simulink library "Contact_Forces_Lib"  (R2024a)
settings: Solver=ode45  StartTime=0.0  StopTime=10.0  RelTol=1e-3  EnableMultiTasking=on
undefined symbols (not defined in the file or in its folder): b_contact, custom_param_1, custom_param_2, Extr_Data_Ring, k_contact, l_cone, length_cylinder, length_tube, mu_kinetic, mu_static, pen_exponent, pen_full_damp_F, rad_s_cone, radius_cylinder, radius_tube, v_thr, X, Y, Z
libraries: nesl_utility x197, sm_lib x115, $bdroot x72, simulink x20, fl_lib x4
(part 11 of 12)

== system Contact_Forces_Lib/3D/Sphere to Cone Force/Forces/Fn/Fn in SphF ==
  R : Inport
  FxConB : Inport  Port=2
  FyConB : Inport  Port=3
  FzConB : Inport  Port=4
  Demux : Demux  Outputs=3
  Divide3 : Product  Inputs=/*  Multiplication=Matrix(*)
  Gain : Gain  Gain=-1
  Mux1 : Mux  Inputs=3
  FySphF : Outport  VectorParamsAs1DForOutWhenUnconnected=off
  FxSphF : Outport  Port=2  VectorParamsAs1DForOutWhenUnconnected=off
  FzSphF : Outport  Port=3  VectorParamsAs1DForOutWhenUnconnected=off
  wires:
  FzConB/1 -> Mux1/3
  Gain/1 -> Demux/1
  R/1 -> Divide3/1
  Demux/1 -> FxSphF/1
  Demux/2 -> FySphF/1
  Demux/3 -> FzSphF/1
  FxConB/1 -> Mux1/1
  FyConB/1 -> Mux1/2
  Mux1/1 -> Divide3/2
  Divide3/1 -> Gain/1

== system Contact_Forces_Lib/3D/Sphere to Cone Force/Forces/Fn/Fn in TubB ==
  Fn : Inport
  azm : Inport  Port=2
  Divide1 : Product  Inputs=**
  Divide2 : Product  Inputs=**
  Gain : Gain  Gain=sinConeTh
  Gain1 : Gain  Gain=sinConeTh
  cos : Trigonometry  Operator=cos
  sin : Trigonometry
  FxConB : Outport  VectorParamsAs1DForOutWhenUnconnected=off
  FyConB : Outport  Port=2  VectorParamsAs1DForOutWhenUnconnected=off
  FzConB : Outport  Port=3  VectorParamsAs1DForOutWhenUnconnected=off
  wires:
  Gain1/1 -> FzConB/1
  Gain/1 -> Divide1/1, Divide2/1
  Fn/1 -> Gain/1, Gain1/1
  azm/1 -> cos/1, sin/1
  sin/1 -> Divide2/2
  cos/1 -> Divide1/2
  Divide1/1 -> FxConB/1
  Divide2/1 -> FyConB/1

== system Contact_Forces_Lib/3D/Sphere to Cone Force/Sensing/rad_azm_cal/rad_0 ==
  Action Port : ActionPort
  Zeros : Constant  Value=[0 0 0 0]  SampleTime=0
  F : Outport  InitialOutput=[0]  VectorParamsAs1DForOutWhenUnconnected=off
  wires:
  Zeros/1 -> F/1

== system Contact_Forces_Lib/3D/Sphere to Cone Force/Sensing/rad_azm_cal/rad_azm_cal ==
  note: vazm = (x*vy - y*vx)/(x^2+y^2)
  note: vrad = (x*vx + y*vy)/z
  note: azm = atan2(y, x)
  note: rad = sqrt(x^2+y^2)
  x : Inport
  y : Inport  Port=2
  vx : Inport  Port=3
  vy : Inport  Port=4
  Action Port : ActionPort
  Add : Sum
  Add1 : Sum  Inputs=+-
  Divide : Product  Inputs=*/
  Divide1 : Product  Inputs=*/
  Math Function : Math  Operator=square  SignedPower=on
  Math Function1 : Math  Operator=square  SignedPower=on
  Mux : Mux
  Product{,1..3} (4 alike) : Product
  Sqrt : Sqrt
  Sum : Sum
  Trigonometric Function : Trigonometry  Operator=atan2
  F : Outport  VectorParamsAs1DForOutWhenUnconnected=off
  wires:
  Math Function1/1 -> Sum/2
  Math Function/1 -> Sum/1
  Sum/1 -> Divide1/2, Sqrt/1
  Trigonometric Function/1 -> Mux/2  "azm"
  x/1 -> Trigonometric Function/2, Product/1, Product2/1, Math Function/1
  y/1 -> Trigonometric Function/1, Product1/1, Product3/1, Math Function1/1
  vx/1 -> Product3/2, Product/2
  vy/1 -> Product2/2, Product1/2
  Product/1 -> Add/1
  Product1/1 -> Add/2
  Add/1 -> Divide/1
  Sqrt/1 -> Mux/1, Divide/2  "rad"
  Divide/1 -> Mux/3  "vrad"
  Product2/1 -> Add1/1
  Product3/1 -> Add1/2
  Add1/1 -> Divide1/1
  Divide1/1 -> Mux/4  "vazm"
  Mux/1 -> F/1

== system Contact_Forces_Lib/3D/Sphere to Cone Force/Sensing/rad_azm_cal/vazmx_0 ==
  Action Port : ActionPort
  Zeros : Constant  Value=0  SampleTime=0
  F : Outport  InitialOutput=[0]  VectorParamsAs1DForOutWhenUnconnected=off
  wires:
  Zeros/1 -> F/1

== system Contact_Forces_Lib/3D/Sphere to Cone Force/Sensing/rad_azm_cal/vazmx_cal ==
  note: vazmx = (y*vz - z*vy)/(y^2+z^2)
  y : Inport
  z : Inport  Port=2
  vy : Inport  Port=3
  vz : Inport  Port=4
  Action Port : ActionPort
  Add2 : Sum  Inputs=+-
  Divide2 : Product  Inputs=*/
  Math Function1 : Math  Operator=square  SignedPower=on
  Math Function2 : Math  Operator=square  SignedPower=on
  Product4 : Product
  Product5 : Product
  Sum1 : Sum
  vazmx : Outport  VectorParamsAs1DForOutWhenUnconnected=off
  wires:
  Product4/1 -> Add2/1
  Product5/1 -> Add2/2
  Add2/1 -> Divide2/1
  vy/1 -> Product5/2
  y/1 -> Math Function1/1, Product4/1
  Math Function1/1 -> Sum1/1
  z/1 -> Product5/1, Math Function2/1
  Math Function2/1 -> Sum1/2
  Sum1/1 -> Divide2/2
  vz/1 -> Product4/2
  Divide2/1 -> vazmx/1  "vazmx"

== system Contact_Forces_Lib/3D/Sphere to Cone Force/Sensing/rad_azm_cal/vazmy_0 ==
  Action Port : ActionPort
  Zeros : Constant  Value=0  SampleTime=0
  F : Outport  InitialOutput=[0]  VectorParamsAs1DForOutWhenUnconnected=off
  wires:
  Zeros/1 -> F/1

== system Contact_Forces_Lib/3D/Sphere to Cone Force/Sensing/rad_azm_cal/vazmy_cal ==
  note: vazmy = (z*vx - x*vz)/(z^2+x^2)
  x : Inport
  z : Inport  Port=2
  vx : Inport  Port=3
  vz : Inport  Port=4
  Action Port : ActionPort
  Add3 : Sum  Inputs=+-
  Divide3 : Product  Inputs=*/
  Math Function : Math  Operator=square  SignedPower=on
  Math Function2 : Math  Operator=square  SignedPower=on
  Product6 : Product
  Product7 : Product
  Sum2 : Sum
  vazmy : Outport  VectorParamsAs1DForOutWhenUnconnected=off
  wires:
  vx/1 -> Product6/2
  x/1 -> Math Function/1, Product7/1
  Math Function/1 -> Sum2/1
  Add3/1 -> Divide3/1
  Product7/1 -> Add3/2
  Product6/1 -> Add3/1
  z/1 -> Product6/1, Math Function2/1
  Math Function2/1 -> Sum2/2
  Sum2/1 -> Divide3/2
  vz/1 -> Product7/2
  Divide3/1 -> vazmy/1  "vazmy"

== system Contact_Forces_Lib/3D/Sphere to Plane Force/Forces/Ff/SlipVel ==
  wx : Inport
  wy : Inport  Port=2
  vx : Inport  Port=3
  vy : Inport  Port=4
  Fx1 : Constant  Value=sphere_rad
  Math Function : Math  Operator=square  SignedPower=on
  Math Function1 : Math  Operator=square  SignedPower=on
  Product3 : Product
  Product4 : Product
  Sqrt : Sqrt
  Sum1 : Sum  Inputs=|++
  Sum2 : Sum  Inputs=|-+
  Sum3 : Sum  Inputs=|++
  Trigonometric Function : Trigonometry  Operator=atan2
  vabs : Outport  VectorParamsAs1DForOutWhenUnconnected=off
  alpha : Outport  Port=2  VectorParamsAs1DForOutWhenUnconnected=off
  wires:
  Sum2/1 -> Math Function1/1, Trigonometric Function/2  "slipx"
  Sum1/1 -> Math Function/1, Trigonometric Function/1  "slipy"
  Math Function1/1 -> Sum3/2
  Math Function/1 -> Sum3/1
  Sum3/1 -> Sqrt/1
  Sqrt/1 -> vabs/1
  Trigonometric Function/1 -> alpha/1
  Product4/1 -> Sum2/1
  vy/1 -> Sum1/2
  Fx1/1 -> Product4/1, Product3/2
  vx/1 -> Sum2/2
  wy/1 -> Product4/2
  Product3/1 -> Sum1/1
  wx/1 -> Product3/1

== system Contact_Forces_Lib/3D/Sphere to Plane Force Enabled/Forces/Ff/SlipVel ==
  wx : Inport
  wy : Inport  Port=2
  vx : Inport  Port=3
  vy : Inport  Port=4
  Fx1 : Constant  Value=sphere_rad
  Math Function : Math  Operator=square  SignedPower=on
  Math Function1 : Math  Operator=square  SignedPower=on
  Product3 : Product
  Product4 : Product
  Sqrt : Sqrt
  Sum1 : Sum  Inputs=|++
  Sum2 : Sum  Inputs=|-+
  Sum3 : Sum  Inputs=|++
  Trigonometric Function : Trigonometry  Operator=atan2
  vabs : Outport  VectorParamsAs1DForOutWhenUnconnected=off
  alpha : Outport  Port=2  VectorParamsAs1DForOutWhenUnconnected=off
  wires:
  wx/1 -> Product3/1
  Product3/1 -> Sum1/1
  wy/1 -> Product4/2
  vx/1 -> Sum2/2
  Fx1/1 -> Product3/2, Product4/1
  vy/1 -> Sum1/2
  Product4/1 -> Sum2/1
  Trigonometric Function/1 -> alpha/1
  Sqrt/1 -> vabs/1
  Sum3/1 -> Sqrt/1
  Math Function/1 -> Sum3/1
  Math Function1/1 -> Sum3/2
  Sum1/1 -> Trigonometric Function/1, Math Function/1  "slipy"
  Sum2/1 -> Trigonometric Function/2, Math Function1/1  "slipx"

== system Contact_Forces_Lib/3D/Sphere to Sphere Force/Ff/Check w or v non zero/Else ==
  Action Port : ActionPort
  Constant : Constant  Value=0  SampleTime=0
  Constant1 : Constant  Value=[0 0 0]  SampleTime=0
  vabs : Outport  InitialOutput=0  VectorParamsAs1DForOutWhenUnconnected=off
  vuvect : Outport  Port=2  InitialOutput=0  VectorParamsAs1DForOutWhenUnconnected=off
  wires:
  Constant1/1 -> vuvect/1
  Constant/1 -> vabs/1

== system Contact_Forces_Lib/3D/Sphere to Sphere Force/Ff/Check w or v non zero/mag v ==
  vect : Inport
  Add2 : Sum  Inputs=+++
  Demux : Demux  Outputs=3
  Math Function : Math  Operator=square  SignedPower=on
  Math Function1 : Math  Operator=square  SignedPower=on
  Math Function2 : Math  Operator=square  SignedPower=on
  Sqrt : Sqrt
  mag : Outport  VectorParamsAs1DForOutWhenUnconnected=off
  wires:
  Demux/2 -> Math Function1/1
  Demux/1 -> Math Function/1
  vect/1 -> Demux/1
  Add2/1 -> Sqrt/1
  Math Function/1 -> Add2/1
  Math Function1/1 -> Add2/2
  Sqrt/1 -> mag/1
  Demux/3 -> Math Function2/1
  Math Function2/1 -> Add2/3

== system Contact_Forces_Lib/3D/Sphere to Sphere Force/Ff/Check w or v non zero/mag w ==
  vect : Inport
  Add : Sum  Inputs=+++
  Demux : Demux  Outputs=3
  Math Function : Math  Operator=square  SignedPower=on
  Math Function1 : Math  Operator=square  SignedPower=on
  Math Function2 : Math  Operator=square  SignedPower=on
  Sqrt : Sqrt
  mag : Outport  VectorParamsAs1DForOutWhenUnconnected=off
  wires:
  Math Function2/1 -> Add/3
  Demux/3 -> Math Function2/1
  Sqrt/1 -> mag/1
  Math Function1/1 -> Add/2
  Math Function/1 -> Add/1
  Add/1 -> Sqrt/1
  vect/1 -> Demux/1
  Demux/1 -> Math Function/1
  Demux/2 -> Math Function1/1

== system Contact_Forces_Lib/3D/Sphere to Sphere Force/Ff/SlipVel/If Action Subsystem ==
  In1 : Inport
  In2 : Inport  Port=2
  Action Port : ActionPort
  Divide : Product  Inputs=/*
  Out1 : Outport  VectorParamsAs1DForOutWhenUnconnected=off
  wires:
  In1/1 -> Divide/1
  In2/1 -> Divide/2
  Divide/1 -> Out1/1

== system Contact_Forces_Lib/3D/Sphere to Sphere Force/Ff/SlipVel/mag ==
  vect : Inport
  Add2 : Sum  Inputs=+++
  Demux : Demux  Outputs=3
  Math Function : Math  Operator=square  SignedPower=on
  Math Function1 : Math  Operator=square  SignedPower=on
  Math Function2 : Math  Operator=square  SignedPower=on
  Sqrt : Sqrt
  mag : Outport  VectorParamsAs1DForOutWhenUnconnected=off
  wires:
  Demux/2 -> Math Function1/1
  Demux/1 -> Math Function/1
  vect/1 -> Demux/1
  Add2/1 -> Sqrt/1
  Math Function/1 -> Add2/1
  Math Function1/1 -> Add2/2
  Sqrt/1 -> mag/1
  Demux/3 -> Math Function2/1
  Math Function2/1 -> Add2/3

== system Contact_Forces_Lib/3D/Sphere to Tube Force/Forces/Ff/Relative vel at CP ==
  note: Calculate relative velocity at contact point between sphere and tube. Two components: about ring and along tube axis. Use magnitude to calculate friction force, atan2 retains relative magnitude and direction between the components.
  Fn : Inport
  rad : Inport  Port=2
  Pen : Inport  Port=3
  vazm : Inport  Port=4
  wzf : Inport  Port=5
  vzf : Inport  Port=6
  wxf : Inport  Port=7
  wyf : Inport  Port=8
  azm : Inport  Port=9
  Calculate vRelAxis : Subsystem
  Calculate vRelRing : Subsystem
  Follower Radius : Constant  Value=radius_sphere
  Math Function : Math  Operator=square  SignedPower=on
  Math Function1 : Math  Operator=square  SignedPower=on
  Midpt Pen : Gain  Gain=0.5
  Product1 : Product
  Sign : Signum  ZeroCross=off
  Sqrt : Sqrt
  Sum1 : Sum  Inputs=+-
  Sum3 : Sum  Inputs=|++
  Trigonometric Function : Trigonometry  Operator=atan2
  vRelAbs : Outport  VectorParamsAs1DForOutWhenUnconnected=off
  rSphtoCP : Outport  Port=2  VectorParamsAs1DForOutWhenUnconnected=off
  rCyltoCP : Outport  Port=3  VectorParamsAs1DForOutWhenUnconnected=off
  alpha : Outport  Port=4  VectorParamsAs1DForOutWhenUnconnected=off
  wires:
  Calculate vRelRing/1(rCyltoCP) -> rCyltoCP/1
  wzf/1 -> Calculate vRelRing/3(wzf)
  vazm/1 -> Calculate vRelRing/2(vazm)
  rad/1 -> Calculate vRelRing/1(rad)
  Calculate vRelRing/2(vRelRing) -> Math Function/1, Trigonometric Function/2  "vRelRing"
  wyf/1 -> Calculate vRelAxis/5(wyf)
  azm/1 -> Calculate vRelAxis/4(azm)
  vzf/1 -> Calculate vRelAxis/3(vzf)
  wxf/1 -> Calculate vRelAxis/2(wxf)
  Calculate vRelAxis/1(vRelAxis) -> Trigonometric Function/1, Math Function1/1  "vRelAxis"
  Midpt Pen/1 -> Sum1/2
  Fn/1 -> Sign/1
  Pen/1 -> Midpt Pen/1
  Follower Radius/1 -> Sum1/1
  Math Function1/1 -> Sum3/2
  Math Function/1 -> Sum3/1
  Sum3/1 -> Sqrt/1
  Sqrt/1 -> vRelAbs/1
  Trigonometric Function/1 -> alpha/1  "alpha"
  Sign/1 -> Product1/2  "InOut"
  Sum1/1 -> Product1/1, rSphtoCP/1  "rSphtoCP"
  Product1/1 -> Calculate vRelAxis/1(rSphtoCP sign), Calculate vRelRing/4(rSphtoCP sign)

== system Contact_Forces_Lib/3D/Sphere to Tube Force/Forces/Ff/Resolve Ff ==
  note: Resolve Friction Force in
      | Tube B reference frame
  note: Resolve Friction Force in
      | Sphere F reference frame
  InOut : Inport
  Ff : Inport  Port=2
  rSphtoCP : Inport  Port=3
  rCyltoCP : Inport  Port=4
  alpha : Inport  Port=5
  z : Inport  Port=6
  R : Inport  Port=7
  azm : Inport  Port=8
  Ff in SphF : Subsystem
  Ff in TubB : Subsystem
  FxSphF : Outport  VectorParamsAs1DForOutWhenUnconnected=off
  FySphF : Outport  Port=2  VectorParamsAs1DForOutWhenUnconnected=off
  FzSphF : Outport  Port=3  VectorParamsAs1DForOutWhenUnconnected=off
  TSphF : Outport  Port=4  VectorParamsAs1DForOutWhenUnconnected=off
  FxSphB : Outport  Port=5  VectorParamsAs1DForOutWhenUnconnected=off
  FyTubB : Outport  Port=6  VectorParamsAs1DForOutWhenUnconnected=off
  FzTubB : Outport  Port=7  VectorParamsAs1DForOutWhenUnconnected=off
  TTubB : Outport  Port=8  VectorParamsAs1DForOutWhenUnconnected=off
  wires:
  InOut/1 -> Ff in TubB/1(InOut)
  z/1 -> Ff in TubB/7(z)
  rSphtoCP/1 -> Ff in TubB/5(rSphtoCP)
  rCyltoCP/1 -> Ff in TubB/6(rCyltoCP)
  Ff/1 -> Ff in TubB/2(Ff)
  Ff in SphF/1(FySphF) -> FySphF/1
  Ff in TubB/1(FxTubB) -> Ff in SphF/1(FxTubB), FxSphB/1
  Ff in TubB/2(FyTubB) -> FyTubB/1, Ff in SphF/2(FyTubB)
  Ff in SphF/2(FxSphF) -> FxSphF/1
  azm/1 -> Ff in TubB/3(azm)
  R/1 -> Ff in SphF/5(R)
  Ff in SphF/3(FzSphF) -> FzSphF/1
  Ff in TubB/3(FzTubB) -> Ff in SphF/3(FzTubB), FzTubB/1
  alpha/1 -> Ff in TubB/4(alpha)
  Ff in TubB/5(TTubB) -> TTubB/1
  Ff in TubB/4(TSphF_B) -> Ff in SphF/4(TSphF_B)
  Ff in SphF/4(TSphF) -> TSphF/1

== system Contact_Forces_Lib/3D/Sphere to Tube Force/Forces/Fn/Fn in SphF ==
  R : Inport
  FxTubB : Inport  Port=2
  FyTubB : Inport  Port=3
  Constant : Constant  Value=0
  Demux : Demux  Outputs=3
  Divide3 : Product  Inputs=/*  Multiplication=Matrix(*)
  Gain : Gain  Gain=-1
  Mux1 : Mux  Inputs=3
  FySphF : Outport  VectorParamsAs1DForOutWhenUnconnected=off
  FxSphF : Outport  Port=2  VectorParamsAs1DForOutWhenUnconnected=off
  FzSphF : Outport  Port=3  VectorParamsAs1DForOutWhenUnconnected=off
  wires:
  Divide3/1 -> Gain/1
  Mux1/1 -> Divide3/2
  FyTubB/1 -> Mux1/2
  FxTubB/1 -> Mux1/1
  Demux/3 -> FzSphF/1
  Demux/2 -> FySphF/1
  Demux/1 -> FxSphF/1
  Constant/1 -> Mux1/3
  R/1 -> Divide3/1
  Gain/1 -> Demux/1

== system Contact_Forces_Lib/3D/Sphere to Tube Force/Forces/Fn/Fn in TubB ==
  Fn : Inport
  azm : Inport  Port=2
  Divide1 : Product  Inputs=**
  Divide2 : Product  Inputs=**
  cos : Trigonometry  Operator=cos
  sin : Trigonometry
  FxTubB : Outport  VectorParamsAs1DForOutWhenUnconnected=off
  FyTubB : Outport  Port=2  VectorParamsAs1DForOutWhenUnconnected=off
  wires:
  Divide2/1 -> FyTubB/1
  Divide1/1 -> FxTubB/1
  cos/1 -> Divide1/2
  sin/1 -> Divide2/2
  azm/1 -> sin/1, cos/1
  Fn/1 -> Divide2/1, Divide1/1

== system Contact_Forces_Lib/3D/Sphere to Tube Force/Sensing/rad_azm_cal/rad_0 ==
  Action Port : ActionPort
  Zeros : Constant  Value=[0 0 0 0]  SampleTime=0
  F : Outport  InitialOutput=[0]  VectorParamsAs1DForOutWhenUnconnected=off
  wires:
  Zeros/1 -> F/1

== system Contact_Forces_Lib/3D/Sphere to Tube Force/Sensing/rad_azm_cal/rad_azm_cal ==
  note: z = sqrt(x2+y2)
      | zdot = 1/z(x*xdot+y*ydot)
      | azm = atan(y/x)
      | azmdot = 1/z2(x*ydot-xdot*y)
  X : Inport
  Y : Inport  Port=2
  Xdot : Inport  Port=3
  Ydot : Inport  Port=4
  Action Port : ActionPort
  Add : Sum
  Add1 : Sum  Inputs=+-
  Divide : Product  Inputs=*/
  Divide1 : Product  Inputs=*/
  Math Function : Math  Operator=square  SignedPower=on
  Math Function1 : Math  Operator=square  SignedPower=on
  Mux : Mux
  Product{,1..3} (4 alike) : Product
  Sqrt : Sqrt
  Sum : Sum  Inputs=|++
  Trigonometric Function : Trigonometry  Operator=atan2
  F : Outport  VectorParamsAs1DForOutWhenUnconnected=off
  wires:
  Mux/1 -> F/1
  Divide1/1 -> Mux/4
  Add1/1 -> Divide1/1
  Product3/1 -> Add1/2
  Product2/1 -> Add1/1
  Divide/1 -> Mux/3
  Sqrt/1 -> Divide/2, Mux/1
  Add/1 -> Divide/1
  Product1/1 -> Add/2
  Product/1 -> Add/1
  Ydot/1 -> Product1/2, Product2/2
  Xdot/1 -> Product/2, Product3/2
  Y/1 -> Math Function1/1, Product1/1, Product3/1, Trigonometric Function/1
  X/1 -> Math Function/1, Product/1, Product2/1, Trigonometric Function/2
  Trigonometric Function/1 -> Mux/2
  Sum/1 -> Sqrt/1, Divide1/2
  Math Function/1 -> Sum/1
  Math Function1/1 -> Sum/2

== system Contact_Forces_Lib/3D/Sphere to Tube Force Enabled/Forces/Ff/Relative vel at CP ==
  note: Calculate relative velocity at contact point between sphere and tube. Two components: about ring and along tube axis. Use magnitude to calculate friction force, atan2 retains relative magnitude and direction between the components.
  Fn : Inport
  rad : Inport  Port=2
  Pen : Inport  Port=3
  vazm : Inport  Port=4
  wzf : Inport  Port=5
  vzf : Inport  Port=6
  wxf : Inport  Port=7
  wyf : Inport  Port=8
  azm : Inport  Port=9
  Calculate vRelAxis : Subsystem
  Calculate vRelRing : Subsystem
  Follower Radius : Constant  Value=radius_sphere
  Math Function : Math  Operator=square  SignedPower=on
  Math Function1 : Math  Operator=square  SignedPower=on
  Midpt Pen : Gain  Gain=0.5
  Product1 : Product
  Sign : Signum  ZeroCross=off
  Sqrt : Sqrt
  Sum1 : Sum  Inputs=+-
  Sum3 : Sum  Inputs=|++
  Trigonometric Function : Trigonometry  Operator=atan2
  vRelAbs : Outport  VectorParamsAs1DForOutWhenUnconnected=off
  rSphtoCP : Outport  Port=2  VectorParamsAs1DForOutWhenUnconnected=off
  rCyltoCP : Outport  Port=3  VectorParamsAs1DForOutWhenUnconnected=off
  alpha : Outport  Port=4  VectorParamsAs1DForOutWhenUnconnected=off
  wires:
  Calculate vRelRing/1(rCyltoCP) -> rCyltoCP/1
  wzf/1 -> Calculate vRelRing/3(wzf)
  vazm/1 -> Calculate vRelRing/2(vazm)
  rad/1 -> Calculate vRelRing/1(rad)
  Calculate vRelRing/2(vRelRing) -> Math Function/1, Trigonometric Function/2  "vRelRing"
  wyf/1 -> Calculate vRelAxis/5(wyf)
  azm/1 -> Calculate vRelAxis/4(azm)
  vzf/1 -> Calculate vRelAxis/3(vzf)
  wxf/1 -> Calculate vRelAxis/2(wxf)
  Calculate vRelAxis/1(vRelAxis) -> Trigonometric Function/1, Math Function1/1  "vRelAxis"
  Midpt Pen/1 -> Sum1/2
  Fn/1 -> Sign/1
  Pen/1 -> Midpt Pen/1
  Follower Radius/1 -> Sum1/1
  Math Function1/1 -> Sum3/2
  Math Function/1 -> Sum3/1
  Sum3/1 -> Sqrt/1
  Sqrt/1 -> vRelAbs/1
  Trigonometric Function/1 -> alpha/1  "alpha"
  Sign/1 -> Product1/2  "InOut"
  Sum1/1 -> Product1/1, rSphtoCP/1  "rSphtoCP"
  Product1/1 -> Calculate vRelAxis/1(rSphtoCP sign), Calculate vRelRing/4(rSphtoCP sign)

== system Contact_Forces_Lib/3D/Sphere to Tube Force Enabled/Forces/Ff/Resolve Ff ==
  note: Resolve Friction Force in
      | Tube B reference frame
  note: Resolve Friction Force in
      | Sphere F reference frame
  InOut : Inport
  Ff : Inport  Port=2
  rSphtoCP : Inport  Port=3
  rCyltoCP : Inport  Port=4
  alpha : Inport  Port=5
  z : Inport  Port=6
  R : Inport  Port=7
  azm : Inport  Port=8
  Ff in SphF : Subsystem
  Ff in TubB : Subsystem
  FxSphF : Outport  VectorParamsAs1DForOutWhenUnconnected=off
  FySphF : Outport  Port=2  VectorParamsAs1DForOutWhenUnconnected=off
  FzSphF : Outport  Port=3  VectorParamsAs1DForOutWhenUnconnected=off
  TSphF : Outport  Port=4  VectorParamsAs1DForOutWhenUnconnected=off
  FxSphB : Outport  Port=5  VectorParamsAs1DForOutWhenUnconnected=off
  FyTubB : Outport  Port=6  VectorParamsAs1DForOutWhenUnconnected=off
  FzTubB : Outport  Port=7  VectorParamsAs1DForOutWhenUnconnected=off
  TTubB : Outport  Port=8  VectorParamsAs1DForOutWhenUnconnected=off
  wires:
  InOut/1 -> Ff in TubB/1(InOut)
  z/1 -> Ff in TubB/7(z)
  rSphtoCP/1 -> Ff in TubB/5(rSphtoCP)
  rCyltoCP/1 -> Ff in TubB/6(rCyltoCP)
  Ff/1 -> Ff in TubB/2(Ff)
  Ff in SphF/1(FySphF) -> FySphF/1
  Ff in TubB/1(FxTubB) -> Ff in SphF/1(FxTubB), FxSphB/1
  Ff in TubB/2(FyTubB) -> FyTubB/1, Ff in SphF/2(FyTubB)
  Ff in SphF/2(FxSphF) -> FxSphF/1
  azm/1 -> Ff in TubB/3(azm)
  R/1 -> Ff in SphF/5(R)
  Ff in SphF/3(FzSphF) -> FzSphF/1
  Ff in TubB/3(FzTubB) -> Ff in SphF/3(FzTubB), FzTubB/1
  alpha/1 -> Ff in TubB/4(alpha)
  Ff in TubB/5(TTubB) -> TTubB/1
  Ff in TubB/4(TSphF_B) -> Ff in SphF/4(TSphF_B)
  Ff in SphF/4(TSphF) -> TSphF/1

== system Contact_Forces_Lib/3D/Sphere to Tube Force Enabled/Forces/Fn/Fn in SphF ==
  R : Inport
  FxTubB : Inport  Port=2
  FyTubB : Inport  Port=3
  Constant : Constant  Value=0
  Demux : Demux  Outputs=3
  Divide3 : Product  Inputs=/*  Multiplication=Matrix(*)
  Gain : Gain  Gain=-1
  Mux1 : Mux  Inputs=3
  FySphF : Outport  VectorParamsAs1DForOutWhenUnconnected=off
  FxSphF : Outport  Port=2  VectorParamsAs1DForOutWhenUnconnected=off
  FzSphF : Outport  Port=3  VectorParamsAs1DForOutWhenUnconnected=off
  wires:
  Divide3/1 -> Gain/1
  Mux1/1 -> Divide3/2
  FyTubB/1 -> Mux1/2
  FxTubB/1 -> Mux1/1
  Demux/3 -> FzSphF/1
  Demux/2 -> FySphF/1
  Demux/1 -> FxSphF/1
  Constant/1 -> Mux1/3
  R/1 -> Divide3/1
  Gain/1 -> Demux/1

== system Contact_Forces_Lib/3D/Sphere to Tube Force Enabled/Forces/Fn/Fn in TubB ==
  Fn : Inport
  azm : Inport  Port=2
  Divide1 : Product  Inputs=**
  Divide2 : Product  Inputs=**
  cos : Trigonometry  Operator=cos
  sin : Trigonometry
  FxTubB : Outport  VectorParamsAs1DForOutWhenUnconnected=off
  FyTubB : Outport  Port=2  VectorParamsAs1DForOutWhenUnconnected=off
  wires:
  Divide2/1 -> FyTubB/1
  Divide1/1 -> FxTubB/1
  cos/1 -> Divide1/2
  sin/1 -> Divide2/2
  azm/1 -> sin/1, cos/1
  Fn/1 -> Divide2/1, Divide1/1

== system Contact_Forces_Lib/3D/Sphere to Tube Force Enabled/Sensing/rad_azm_cal/rad_0 ==
  Action Port : ActionPort
  Zeros : Constant  Value=[0 0 0 0]  SampleTime=0
  F : Outport  InitialOutput=[0]  VectorParamsAs1DForOutWhenUnconnected=off
  wires:
  Zeros/1 -> F/1

== system Contact_Forces_Lib/3D/Sphere to Tube Force Enabled/Sensing/rad_azm_cal/rad_azm_cal ==
  note: z = sqrt(x2+y2)
      | zdot = 1/z(x*xdot+y*ydot)
      | azm = atan(y/x)
      | azmdot = 1/z2(x*ydot-xdot*y)
  X : Inport
  Y : Inport  Port=2
  Xdot : Inport  Port=3
  Ydot : Inport  Port=4
  Action Port : ActionPort
  Add : Sum
  Add1 : Sum  Inputs=+-
  Divide : Product  Inputs=*/
  Divide1 : Product  Inputs=*/
  Math Function : Math  Operator=square  SignedPower=on
  Math Function1 : Math  Operator=square  SignedPower=on
  Mux : Mux
  Product{,1..3} (4 alike) : Product
  Sqrt : Sqrt
  Sum : Sum  Inputs=|++
  Trigonometric Function : Trigonometry  Operator=atan2
  F : Outport  VectorParamsAs1DForOutWhenUnconnected=off
  wires:
  Mux/1 -> F/1
  Divide1/1 -> Mux/4
  Add1/1 -> Divide1/1
  Product3/1 -> Add1/2
  Product2/1 -> Add1/1
  Divide/1 -> Mux/3
  Sqrt/1 -> Divide/2, Mux/1
  Add/1 -> Divide/1
  Product1/1 -> Add/2
  Product/1 -> Add/1
  Ydot/1 -> Product1/2, Product2/2
  Xdot/1 -> Product/2, Product3/2
  Y/1 -> Math Function1/1, Product1/1, Product3/1, Trigonometric Function/1
  X/1 -> Math Function/1, Product/1, Product2/1, Trigonometric Function/2
  Trigonometric Function/1 -> Mux/2
  Sum/1 -> Sqrt/1, Divide1/2
  Math Function/1 -> Sum/1
  Math Function1/1 -> Sum/2

== system Contact_Forces_Lib/2D/Circle to Finite Line Force/Forces/Resolve Forces/Friction/VCirPt ==
  wz : Inport
  X sep : Inport  Port=2
  Constant : Constant  Value=line_depth
  Product : Product
  Product1 : Product
  Sign1 : Signum
  Subtract : Sum  Inputs=+-
  vCir : Outport  VectorParamsAs1DForOutWhenUnconnected=off
  wires:
  wz/1 -> Product1/1
  Product1/1 -> vCir/1
  Product/1 -> Subtract/2
  Sign1/1 -> Product/1
  X sep/1 -> Subtract/1, Sign1/1
  Constant/1 -> Product/2
  Subtract/1 -> Product1/2

== system Contact_Forces_Lib/2D/Circle to Finite Line Force Enabled/Forces/Resolve Forces/Friction/VCirPt ==
  wz : Inport
  X sep : Inport  Port=2
  Constant : Constant  Value=line_depth
  Product : Product
  Product1 : Product
  Sign1 : Signum
  Subtract : Sum  Inputs=+-
  vCir : Outport  VectorParamsAs1DForOutWhenUnconnected=off
  wires:
  Subtract/1 -> Product1/2
  Constant/1 -> Product/2
  X sep/1 -> Sign1/1, Subtract/1
  Sign1/1 -> Product/1
  Product/1 -> Subtract/2
  Product1/1 -> vCir/1
  wz/1 -> Product1/1

== system Contact_Forces_Lib/2D/Circle to Ring Force/Forces/Ff/Resolve Ff/Ff in CirB ==
  Ff : Inport
  azm : Inport  Port=2
  Divide1 : Product  Inputs=**
  Divide2 : Product  Inputs=**
  Gain1 : Gain
  Gain3 : Gain  Gain=-1
  cos : Trigonometry
  deg2rad : Gain  Gain=pi/180
  sin : Trigonometry  Operator=cos
  FxRinB : Outport  VectorParamsAs1DForOutWhenUnconnected=off
  FyRinB : Outport  Port=2  VectorParamsAs1DForOutWhenUnconnected=off
  wires:
  Gain1/1 -> Divide2/1, Divide1/1
  azm/1 -> deg2rad/1
  Divide2/1 -> FyRinB/1
  cos/1 -> Gain3/1
  sin/1 -> Divide2/2
  deg2rad/1 -> sin/1, cos/1
  Divide1/1 -> FxRinB/1
  Ff/1 -> Gain1/1
  Gain3/1 -> Divide1/2

== system Contact_Forces_Lib/2D/Circle to Ring Force/Forces/Ff/Resolve Ff/Ff in CirF ==
  R : Inport
  FxRinB : Inport  Port=2
  FyRinB : Inport  Port=3
  Demux : Demux  Outputs=2
  Divide3 : Product  Inputs=**  Multiplication=Matrix(*)
  Gain1 : Gain  Gain=-1
  Mux1 : Mux  Inputs=2
  FyCirF : Outport  VectorParamsAs1DForOutWhenUnconnected=off
  FxCirF : Outport  Port=2  VectorParamsAs1DForOutWhenUnconnected=off
  wires:
  R/1 -> Divide3/1
  Divide3/1 -> Gain1/1
  Mux1/1 -> Divide3/2
  Gain1/1 -> Demux/1
  Demux/1 -> FyCirF/1
  Demux/2 -> FxCirF/1
  FyRinB/1 -> Mux1/1
  FxRinB/1 -> Mux1/2

== system Contact_Forces_Lib/2D/Circle to Ring Force/Forces/Ff/Resolve Ff/Tz ==
  rCirFtoCP : Inport
  rRinBtoCP : Inport  Port=2
  Ff : Inport  Port=3
  Divide4 : Product  Inputs=**
  Divide5 : Product  Inputs=**
  Gain2 : Gain  Gain=-1
  TzRinB : Outport  VectorParamsAs1DForOutWhenUnconnected=off
  TzCirF : Outport  Port=2  VectorParamsAs1DForOutWhenUnconnected=off
  wires:
  rRinBtoCP/1 -> Divide5/2
  Divide5/1 -> TzRinB/1
  rCirFtoCP/1 -> Divide4/2
  Divide4/1 -> TzCirF/1
  Gain2/1 -> Divide5/1
  Ff/1 -> Divide4/1, Gain2/1

== system Contact_Forces_Lib/3D/Prototype/Cone in Ring Force/Point of Contact calc/Force Calc/Computing Force from nonzero penetration points ==
  Y : Inport
  X : Inport  Port=2
  Pen : Inport  Port=3
  Derivative : Derivative  Commented=on  CoefficientInTFapproximation=1e-4
  For Each Subsystem1 : Subsystem  Commented=on  TreatAsAtomicUnit=on
  For Iterator Subsystem : Subsystem  Commented=on  TreatAsAtomicUnit=on
  Gain1 : Gain  Commented=on  Gain=-1
  Linear1 : Subsystem  Commented=on  VariantControl=Linear  mask(Linear Force Law){k_pen=1e4, b_penvel=1e3}
      mask prompts: k_pen "Contact Stiffness"; b_penvel "Contact Damping"
      mask help: Implements a contact force law as a linear spring damper. The damping force is applied only as the penetration depth increases.
      mask Help: web(which('Force_Laws.html'));
  Product2 : Product  Commented=on
  Product3 : Product  Commented=on
  Sum of Elements : Sum  Commented=on  Inputs=+
  Sum of Elements1 : Sum  Commented=on  Inputs=+
  Sum3 : Sum  Commented=on  Inputs=|+-
  Trigonometric Function3 : Trigonometry  Commented=on  Operator=atan2
  Trigonometric Function4 : Trigonometry  Commented=on  Operator=cos
  Trigonometric Function5 : Trigonometry  Commented=on
  Fx : Outport  VectorParamsAs1DForOutWhenUnconnected=off
  Fy : Outport  Port=2  VectorParamsAs1DForOutWhenUnconnected=off
  wires:
  Trigonometric Function3/1 -> Trigonometric Function5/1, Trigonometric Function4/1
  Linear1/2(Damp F) -> Sum3/2
  Trigonometric Function5/1 -> Product3/1
  Trigonometric Function4/1 -> Product2/1
  Gain1/1 -> Product2/2, Product3/2
  Sum3/1 -> Gain1/1
  Linear1/1(Spr F) -> Sum3/1
  Sum of Elements1/1 -> Fy/1
  Pen/1 -> Derivative/1, For Each Subsystem1/1(In1), Linear1/1(Pen)
  X/1 -> Trigonometric Function3/2
  Y/1 -> Trigonometric Function3/1
  Sum of Elements/1 -> Fx/1
  Derivative/1 -> Linear1/2(Pen Vel)
  Product2/1 -> Sum of Elements/1
  Product3/1 -> Sum of Elements1/1

== system Contact_Forces_Lib/3D/Prototype/Cone in Ring Force/Point of Contact calc/Force Calc/MAX_ML ==
  Y : Inport
  X : Inport  Port=2
  pen : Inport  Port=3
  Gain : Gain  Gain=-1
  Linear : Subsystem  VariantControl=Linear  mask(Linear Force Law){k_pen=k_stiff, b_penvel=b_damp}
      mask prompts: k_pen "Contact Stiffness"; b_penvel "Contact Damping"
      mask help: Implements a contact force law as a linear spring damper. The damping force is applied only as the penetration depth increases.
      mask Help: web(which('Force_Laws.html'));
  MATLAB Function : MATLAB Function  TreatAsAtomicUnit=on
  Product : Product
  Product1 : Product
  Sum2 : Sum  Inputs=|+-
  Transfer Fcn : TransferFcn  Numerator=[1 0]  Denominator=[1e-4 1]
  Trigonometric Function : Trigonometry  Operator=atan2
  Trigonometric Function1 : Trigonometry  Operator=cos
  Trigonometric Function2 : Trigonometry
  Fx : Outport  VectorParamsAs1DForOutWhenUnconnected=off
  Fy : Outport  Port=2  VectorParamsAs1DForOutWhenUnconnected=off
  wires:
  Product1/1 -> Fy/1
  MATLAB Function/4(ind) -> ?
  X/1 -> MATLAB Function/2(x)
  Product/1 -> Fx/1
  pen/1 -> MATLAB Function/1(pen)
  Transfer Fcn/1 -> Linear/2(Pen Vel)
  Gain/1 -> Product1/2, Product/2
  Trigonometric Function1/1 -> Product/1
  Linear/1(Spr F) -> Sum2/1
  Trigonometric Function2/1 -> Product1/1
  Sum2/1 -> Gain/1
  Linear/2(Damp F) -> Sum2/2
  Trigonometric Function/1 -> Trigonometric Function1/1, Trigonometric Function2/1
  Y/1 -> MATLAB Function/3(y)
  MATLAB Function/2(yc) -> Trigonometric Function/1
  MATLAB Function/1(xc) -> Trigonometric Function/2
  MATLAB Function/3(penc) -> Transfer Fcn/1, Linear/1(Pen)

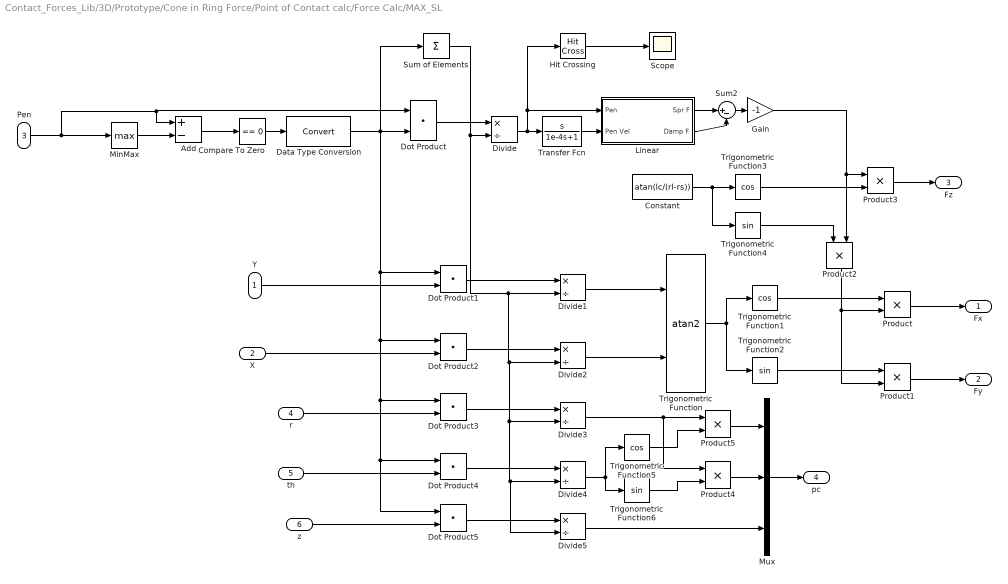
== system Contact_Forces_Lib/3D/Prototype/Cone in Ring Force/Point of Contact calc/Force Calc/MAX_SL ==
  Y : Inport
  X : Inport  Port=2
  Pen : Inport  Port=3
  r : Inport  Port=4
  th : Inport  Port=5
  z : Inport  Port=6
  Add : Sum  Inputs=+-
  Compare To Zero : simulink/Logic and Bit Operations/Compare To Zero  relop===  OutDataTypeStr=boolean  ZeroCross=off
  Constant : Constant  Value=atan(lc/(rl-rs))
  Data Type Conversion : DataTypeConversion  SaturateOnIntegerOverflow=off  RndMeth=Floor
  Divide{,1..5} (6 alike) : Product  Inputs=*/
  Dot Product{,1..5} (6 alike) : DotProduct  OutDataTypeStr=Inherit: Inherit via internal rule
  Gain : Gain  Gain=-1
  Hit Crossing : HitCross
  Linear : Subsystem  VariantControl=Linear  mask(Linear Force Law){k_pen=k_stiff, b_penvel=b_damp}
      mask prompts: k_pen "Contact Stiffness"; b_penvel "Contact Damping"
      mask help: Implements a contact force law as a linear spring damper. The damping force is applied only as the penetration depth increases.
      mask Help: web(which('Force_Laws.html'));
  MinMax : MinMax  Function=max  ZeroCross=off
  Mux : Mux  Inputs=3
  Product{,1..5} (6 alike) : Product
  Scope : Scope
  Sum of Elements : Sum  Inputs=+
  Sum2 : Sum  Inputs=|+-
  Transfer Fcn : TransferFcn  Numerator=[1 0]  Denominator=[1e-4 1]
  Trigonometric Function : Trigonometry  Operator=atan2
  Trigonometric Function1 : Trigonometry  Operator=cos
  Trigonometric Function2 : Trigonometry
  Trigonometric Function3 : Trigonometry  Operator=cos
  Trigonometric Function4 : Trigonometry
  Trigonometric Function5 : Trigonometry  Operator=cos
  Trigonometric Function6 : Trigonometry
  Fx : Outport  VectorParamsAs1DForOutWhenUnconnected=off
  Fy : Outport  Port=2  VectorParamsAs1DForOutWhenUnconnected=off
  Fz : Outport  Port=3  VectorParamsAs1DForOutWhenUnconnected=off
  pc : Outport  Port=4  VectorParamsAs1DForOutWhenUnconnected=off
  wires:
  Trigonometric Function/1 -> Trigonometric Function2/1, Trigonometric Function1/1
  Linear/2(Damp F) -> Sum2/2
  Sum2/1 -> Gain/1
  Trigonometric Function2/1 -> Product1/1
  Linear/1(Spr F) -> Sum2/1
  Trigonometric Function1/1 -> Product/1
  Transfer Fcn/1 -> Linear/2(Pen Vel)
  MinMax/1 -> Add/2
  Add/1 -> Compare To Zero/1
  Compare To Zero/1 -> Data Type Conversion/1
  Product/1 -> Fx/1
  Pen/1 -> Dot Product/1, Add/1, MinMax/1
  Product1/1 -> Fy/1
  Y/1 -> Dot Product1/2
  X/1 -> Dot Product2/2
  Data Type Conversion/1 -> Dot Product/2, Dot Product1/1, Dot Product5/1, Dot Product4/1, Dot Product3/1, Dot Product2/1, Sum of Elements/1
  Dot Product/1 -> Divide/1
  Sum of Elements/1 -> Divide1/2, Divide5/2, Divide4/2, Divide3/2, Divide2/2, Divide/2
  Dot Product1/1 -> Divide1/1
  Dot Product2/1 -> Divide2/1
  Divide1/1 -> Trigonometric Function/1
  Divide2/1 -> Trigonometric Function/2
  Divide/1 -> Hit Crossing/1, Linear/1(Pen), Transfer Fcn/1
  Hit Crossing/1 -> Scope/1
  Constant/1 -> Trigonometric Function4/1, Trigonometric Function3/1
  Trigonometric Function4/1 -> Product2/1
  Gain/1 -> Product3/1, Product2/2
  Product2/1 -> Product1/2, Product/2
  Product3/1 -> Fz/1
  Trigonometric Function3/1 -> Product3/2
  Mux/1 -> pc/1
  Dot Product3/1 -> Divide3/1
  Dot Product4/1 -> Divide4/1
  Dot Product5/1 -> Divide5/1
  r/1 -> Dot Product3/2
  th/1 -> Dot Product4/2
  z/1 -> Dot Product5/2
  Divide5/1 -> Mux/3
  Product4/1 -> Mux/2
  Product5/1 -> Mux/1
  Divide4/1 -> Trigonometric Function5/1, Trigonometric Function6/1
  Divide3/1 -> Product4/1, Product5/1
  Trigonometric Function5/1 -> Product5/2
  Trigonometric Function6/1 -> Product4/2

== system Contact_Forces_Lib/3D/Prototype/Cylinder In Ring Force/Point of Contact calc/Force Calc/Computing Force from nonzero penetration points ==
  Y : Inport
  X : Inport  Port=2
  Pen : Inport  Port=3
  Derivative : Derivative  Commented=on  CoefficientInTFapproximation=1e-4
  For Each Subsystem1 : Subsystem  Commented=on  TreatAsAtomicUnit=on
  For Iterator Subsystem : Subsystem  Commented=on  TreatAsAtomicUnit=on
  Gain1 : Gain  Commented=on  Gain=-1
  Linear1 : Subsystem  Commented=on  VariantControl=Linear  mask(Linear Force Law){k_pen=1e4, b_penvel=1e3}
      mask prompts: k_pen "Contact Stiffness"; b_penvel "Contact Damping"
      mask help: Implements a contact force law as a linear spring damper. The damping force is applied only as the penetration depth increases.
      mask Help: web(which('Force_Laws.html'));
  Product2 : Product  Commented=on
  Product3 : Product  Commented=on
  Sum of Elements : Sum  Commented=on  Inputs=+
  Sum of Elements1 : Sum  Commented=on  Inputs=+
  Sum3 : Sum  Commented=on  Inputs=|+-
  Trigonometric Function3 : Trigonometry  Commented=on  Operator=atan2
  Trigonometric Function4 : Trigonometry  Commented=on  Operator=cos
  Trigonometric Function5 : Trigonometry  Commented=on
  Fx : Outport  VectorParamsAs1DForOutWhenUnconnected=off
  Fy : Outport  Port=2  VectorParamsAs1DForOutWhenUnconnected=off
  wires:
  Trigonometric Function3/1 -> Trigonometric Function5/1, Trigonometric Function4/1
  Linear1/2(Damp F) -> Sum3/2
  Trigonometric Function5/1 -> Product3/1
  Trigonometric Function4/1 -> Product2/1
  Gain1/1 -> Product2/2, Product3/2
  Sum3/1 -> Gain1/1
  Linear1/1(Spr F) -> Sum3/1
  Sum of Elements1/1 -> Fy/1
  Pen/1 -> Derivative/1, For Each Subsystem1/1(In1), Linear1/1(Pen)
  X/1 -> Trigonometric Function3/2
  Y/1 -> Trigonometric Function3/1
  Sum of Elements/1 -> Fx/1
  Derivative/1 -> Linear1/2(Pen Vel)
  Product2/1 -> Sum of Elements/1
  Product3/1 -> Sum of Elements1/1

== system Contact_Forces_Lib/3D/Prototype/Cylinder In Ring Force/Point of Contact calc/Force Calc/MAX_ML ==
  Y : Inport
  X : Inport  Port=2
  pen : Inport  Port=3
  Gain : Gain  Gain=-1
  Linear : Subsystem  VariantControl=Linear  mask(Linear Force Law){k_pen=1e5, b_penvel=1e3}
      mask prompts: k_pen "Contact Stiffness"; b_penvel "Contact Damping"
      mask help: Implements a contact force law as a linear spring damper. The damping force is applied only as the penetration depth increases.
      mask Help: web(which('Force_Laws.html'));
  MATLAB Function : MATLAB Function  TreatAsAtomicUnit=on
  Product : Product
  Product1 : Product
  Sum2 : Sum  Inputs=|+-
  Transfer Fcn : TransferFcn  Numerator=[1 0]  Denominator=[1e-4 1]
  Trigonometric Function : Trigonometry  Operator=atan2
  Trigonometric Function1 : Trigonometry  Operator=cos
  Trigonometric Function2 : Trigonometry
  Fx : Outport  VectorParamsAs1DForOutWhenUnconnected=off
  Fy : Outport  Port=2  VectorParamsAs1DForOutWhenUnconnected=off
  wires:
  Product1/1 -> Fy/1
  MATLAB Function/4(ind) -> ?
  X/1 -> MATLAB Function/2(x)
  Product/1 -> Fx/1
  pen/1 -> MATLAB Function/1(pen)
  Transfer Fcn/1 -> Linear/2(Pen Vel)
  Gain/1 -> Product1/2, Product/2
  Trigonometric Function1/1 -> Product/1
  Linear/1(Spr F) -> Sum2/1
  Trigonometric Function2/1 -> Product1/1
  Sum2/1 -> Gain/1
  Linear/2(Damp F) -> Sum2/2
  Trigonometric Function/1 -> Trigonometric Function1/1, Trigonometric Function2/1
  Y/1 -> MATLAB Function/3(y)
  MATLAB Function/2(yc) -> Trigonometric Function/1
  MATLAB Function/1(xc) -> Trigonometric Function/2
  MATLAB Function/3(penc) -> Transfer Fcn/1, Linear/1(Pen)

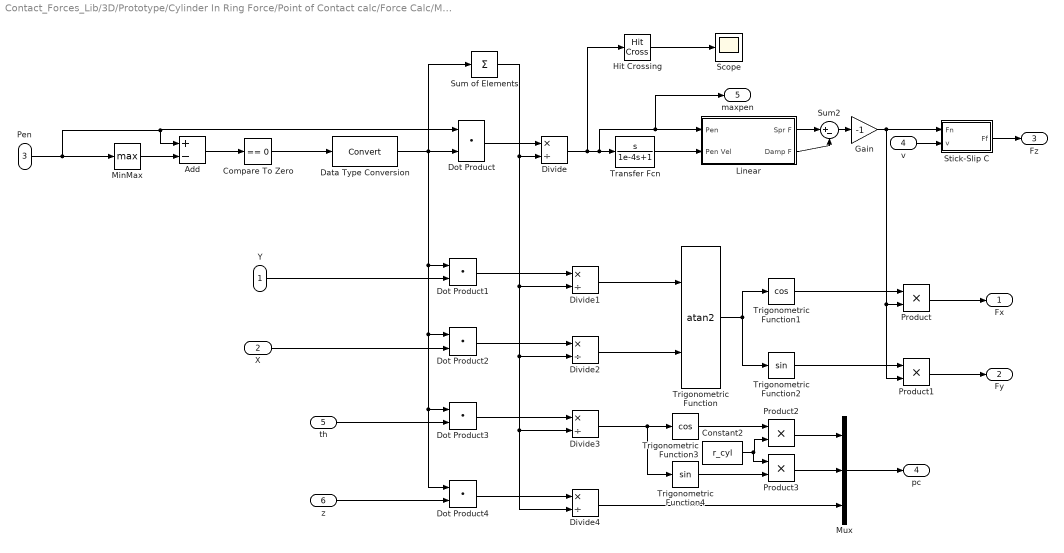
== system Contact_Forces_Lib/3D/Prototype/Cylinder In Ring Force/Point of Contact calc/Force Calc/MAX_SL ==
  Y : Inport
  X : Inport  Port=2
  Pen : Inport  Port=3
  v : Inport  Port=4
  th : Inport  Port=5
  z : Inport  Port=6
  Add : Sum  Inputs=+-
  Compare To Zero : simulink/Logic and Bit Operations/Compare To Zero  relop===  OutDataTypeStr=boolean  ZeroCross=off
  Constant2 : Constant  Value=r_cyl
  Data Type Conversion : DataTypeConversion  SaturateOnIntegerOverflow=off  RndMeth=Floor
  Divide{,1..4} (5 alike) : Product  Inputs=*/
  Dot Product{,1..4} (5 alike) : DotProduct  OutDataTypeStr=Inherit: Inherit via internal rule
  Gain : Gain  Gain=-1
  Hit Crossing : HitCross
  Linear : Subsystem  VariantControl=Linear  mask(Linear Force Law){k_pen=k_stiff, b_penvel=b_damp}
      mask prompts: k_pen "Contact Stiffness"; b_penvel "Contact Damping"
      mask help: Implements a contact force law as a linear spring damper. The damping force is applied only as the penetration depth increases.
      mask Help: web(which('Force_Laws.html'));
  MinMax : MinMax  Function=max  ZeroCross=off
  Mux : Mux  Inputs=3
  Product{,1..3} (4 alike) : Product
  Scope : Scope
  "Stick-Slip C " : Subsystem  VariantControl=Stick_Slip_C  mask(Stick-Slip Friction, Continuous){muk=mu_kinetic, mus=mu_static, vth=v_thr}
      mask prompts: muk "Coefficient of Kinetic Friction"; mus "Coefficient of Static Friction"; vth "Velocity Threshold"
      mask help: Implements a continuous stick-slip friction model. Smaller velocity threshold is closer to reality but results in a numerically stiffer system.
  Sum of Elements : Sum  Inputs=+
  Sum2 : Sum  Inputs=|+-
  Transfer Fcn : TransferFcn  Numerator=[1 0]  Denominator=[1e-4 1]
  Trigonometric Function : Trigonometry  Operator=atan2
  Trigonometric Function1 : Trigonometry  Operator=cos
  Trigonometric Function2 : Trigonometry
  Trigonometric Function3 : Trigonometry  Operator=cos
  Trigonometric Function4 : Trigonometry
  Fx : Outport  VectorParamsAs1DForOutWhenUnconnected=off
  Fy : Outport  Port=2  VectorParamsAs1DForOutWhenUnconnected=off
  Fz : Outport  Port=3  VectorParamsAs1DForOutWhenUnconnected=off
  pc : Outport  Port=4  VectorParamsAs1DForOutWhenUnconnected=off
  maxpen : Outport  Port=5  VectorParamsAs1DForOutWhenUnconnected=off
  wires:
  Trigonometric Function/1 -> Trigonometric Function2/1, Trigonometric Function1/1
  Linear/2(Damp F) -> Sum2/2
  Sum2/1 -> Gain/1
  Trigonometric Function2/1 -> Product1/1
  Linear/1(Spr F) -> Sum2/1
  Trigonometric Function1/1 -> Product/1
  Gain/1 -> "Stick-Slip C "/1(Fn), Product1/2, Product/2
  Transfer Fcn/1 -> Linear/2(Pen Vel)
  MinMax/1 -> Add/2
  Add/1 -> Compare To Zero/1
  Compare To Zero/1 -> Data Type Conversion/1
  Product/1 -> Fx/1
  Pen/1 -> Dot Product/1, Add/1, MinMax/1
  Product1/1 -> Fy/1
  Y/1 -> Dot Product1/2
  X/1 -> Dot Product2/2
  Data Type Conversion/1 -> Dot Product/2, Dot Product4/1, Dot Product3/1, Dot Product2/1, Dot Product1/1, Sum of Elements/1
  Dot Product/1 -> Divide/1
  Sum of Elements/1 -> Divide1/2, Divide4/2, Divide3/2, Divide2/2, Divide/2
  Divide/1 -> Hit Crossing/1, maxpen/1, Linear/1(Pen), Transfer Fcn/1
  Dot Product1/1 -> Divide1/1
  Dot Product2/1 -> Divide2/1
  Divide1/1 -> Trigonometric Function/1
  Divide2/1 -> Trigonometric Function/2
  Hit Crossing/1 -> Scope/1
  v/1 -> "Stick-Slip C "/2(v)
  Dot Product3/1 -> Divide3/1
  Dot Product4/1 -> Divide4/1
  th/1 -> Dot Product3/2
  z/1 -> Dot Product4/2
  Divide3/1 -> Trigonometric Function4/1, Trigonometric Function3/1
  Trigonometric Function3/1 -> Product2/1
  Trigonometric Function4/1 -> Product3/2
  Constant2/1 -> Product3/1, Product2/2
  Product2/1 -> Mux/1
  Product3/1 -> Mux/2
  Divide4/1 -> Mux/3
  "Stick-Slip C "/1(Ff) -> Fz/1
  Mux/1 -> pc/1

== system Contact_Forces_Lib/3D/Sphere to Cone Force/Forces/Ff/Relative vel at CP/Calculate vRelFace ==
  rSphtoCP sign : Inport
  azm : Inport  Port=2
  wxf : Inport  Port=3
  wyf : Inport  Port=4
  vzf : Inport  Port=5
  vrad : Inport  Port=6
  Gain : Gain  Gain=cosConeTh
  Gain{1..2,4..5} (4 alike) : Gain  Gain=-1
  Gain3 : Gain  Gain=sinConeTh
  Product : Product
  Product1 : Product
  Product2 : Product
  Sum : Sum
  Sum1 : Sum
  Sum3 : Sum
  Trigonometric Function3 : Trigonometry  Operator=cos
  Trigonometric Function4 : Trigonometry
  vRelFace : Outport  VectorParamsAs1DForOutWhenUnconnected=off
  wires:
  Gain4/1 -> Sum3/2  "vFaceTra"
  Gain5/1 -> Sum1/1
  Gain3/1 -> Gain5/1
  vzf/1 -> Gain3/1
  Gain/1 -> Sum1/2
  vrad/1 -> Gain/1
  Gain1/1 -> Product2/1
  Gain2/1 -> Sum/2  "wyCP"
  Trigonometric Function4/1 -> Product/1
  Product1/1 -> Gain2/1
  Sum3/1 -> vRelFace/1  "vRelFace"
  wyf/1 -> Product1/2
  Sum/1 -> Product2/2  "wxyzCP"
  rSphtoCP sign/1 -> Gain1/1
  Sum1/1 -> Gain4/1
  Product/1 -> Sum/1  "wxCP"
  wxf/1 -> Product/2
  Trigonometric Function3/1 -> Product1/1
  Product2/1 -> Sum3/1  "vFaceRot"
  azm/1 -> Trigonometric Function3/1, Trigonometric Function4/1

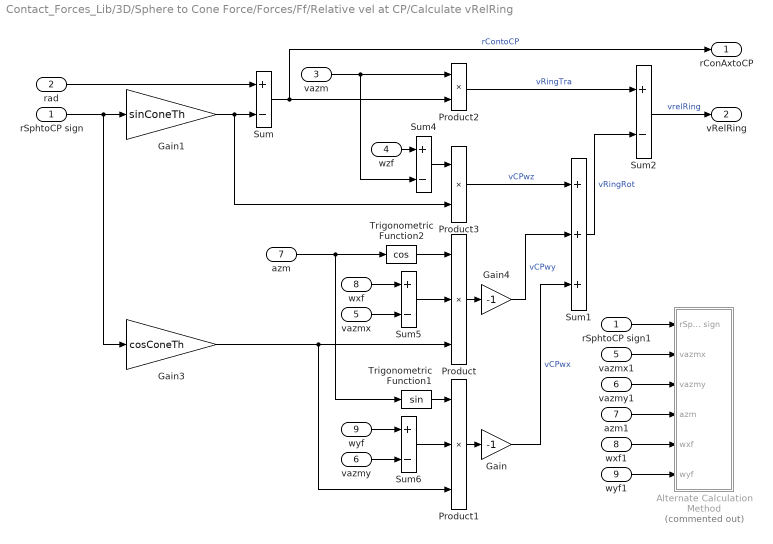
== system Contact_Forces_Lib/3D/Sphere to Cone Force/Forces/Ff/Relative vel at CP/Calculate vRelRing ==
  rSphtoCP sign : Inport
  rad : Inport  Port=2
  vazm : Inport  Port=3
  wzf : Inport  Port=4
  vazmx : Inport  Port=5
  vazmy : Inport  Port=6
  azm : Inport  Port=7
  wxf : Inport  Port=8
  wyf : Inport  Port=9
  Alternate Calculation Method : Subsystem  Commented=on
  Gain : Gain  Gain=-1
  Gain1 : Gain  Gain=sinConeTh
  Gain3 : Gain  Gain=cosConeTh
  Gain4 : Gain  Gain=-1
  Product : Product  Inputs=3
  Product1 : Product  Inputs=3
  Product2 : Product
  Product3 : Product
  Sum{,2,4..6} (5 alike) : Sum  Inputs=+-
  Sum1 : Sum  Inputs=+++
  Trigonometric Function1 : Trigonometry
  Trigonometric Function2 : Trigonometry  Operator=cos
  azm1 : InportShadow  Port=7
  rSphtoCP sign1 : InportShadow
  vazmx1 : InportShadow  Port=5
  vazmy1 : InportShadow  Port=6
  wxf1 : InportShadow  Port=8
  wyf1 : InportShadow  Port=9
  rConAxtoCP : Outport  VectorParamsAs1DForOutWhenUnconnected=off
  vRelRing : Outport  Port=2  VectorParamsAs1DForOutWhenUnconnected=off
  wires:
  wyf1/1 -> Alternate Calculation Method/6(wyf)
  wxf1/1 -> Alternate Calculation Method/5(wxf)
  azm1/1 -> Alternate Calculation Method/4(azm)
  vazmy1/1 -> Alternate Calculation Method/3(vazmy)
  vazmx1/1 -> Alternate Calculation Method/2(vazmx)
  rSphtoCP sign1/1 -> Alternate Calculation Method/1(rSphtoCP sign)
  Gain4/1 -> Sum1/2  "vCPwy"
  Sum6/1 -> Product1/2
  vazmy/1 -> Sum6/2
  wyf/1 -> Sum6/1
  vazmx/1 -> Sum5/2
  wxf/1 -> Sum5/1
  Product3/1 -> Sum1/1  "vCPwz"
  Gain3/1 -> Product1/3, Product/3
  Gain/1 -> Sum1/3  "vCPwx"
  Product1/1 -> Gain/1
  Trigonometric Function1/1 -> Product1/1
  Sum5/1 -> Product/2
  azm/1 -> Trigonometric Function1/1, Trigonometric Function2/1
  Product/1 -> Gain4/1
  Trigonometric Function2/1 -> Product/1
  Gain1/1 -> Sum/2, Product3/2
  rSphtoCP sign/1 -> Gain3/1, Gain1/1
  rad/1 -> Sum/1
  wzf/1 -> Sum4/1
  vazm/1 -> Product2/1, Sum4/2
  Product2/1 -> Sum2/1  "vRingTra"
  Sum/1 -> rConAxtoCP/1, Product2/2  "rContoCP"
  Sum2/1 -> vRelRing/1  "vrelRing"
  Sum1/1 -> Sum2/2  "vRingRot"
  Sum4/1 -> Product3/1

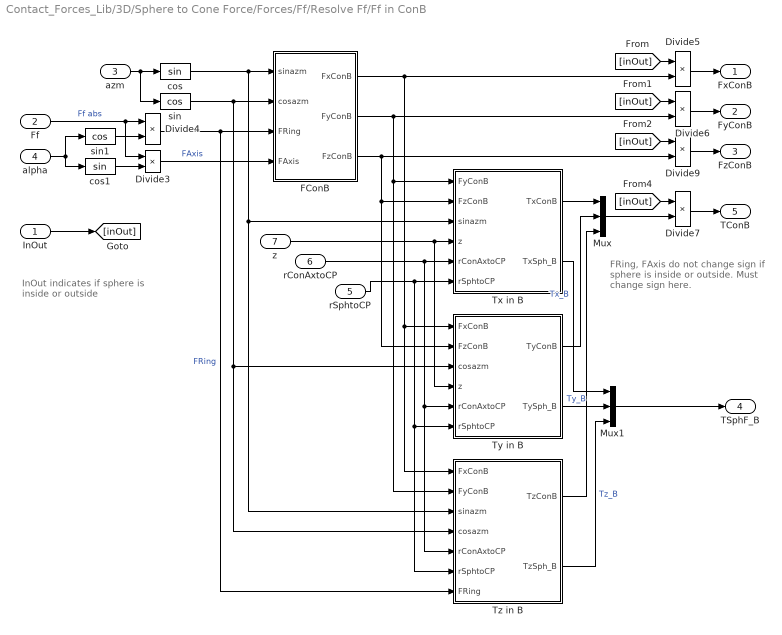
== system Contact_Forces_Lib/3D/Sphere to Cone Force/Forces/Ff/Resolve Ff/Ff in ConB ==
  note: InOut indicates if sphere is inside or outside
  note: FRing, FAxis do not change sign if sphere is inside or outside. Must change sign here.
  InOut : Inport
  Ff : Inport  Port=2
  azm : Inport  Port=3
  alpha : Inport  Port=4
  rSphtoCP : Inport  Port=5
  rConAxtoCP : Inport  Port=6
  z : Inport  Port=7
  Divide{3..7,9} (6 alike) : Product  Inputs=**
  FConB : Subsystem
  Mux : Mux  Inputs=3
  Mux1 : Mux  Inputs=3
  Tx in B : Subsystem
  Ty in B : Subsystem
  Tz in B : Subsystem
  cos : Trigonometry
  cos1 : Trigonometry
  sin : Trigonometry  Operator=cos
  sin1 : Trigonometry  Operator=cos
  FxConB : Outport  VectorParamsAs1DForOutWhenUnconnected=off
  FyConB : Outport  Port=2  VectorParamsAs1DForOutWhenUnconnected=off
  FzConB : Outport  Port=3  VectorParamsAs1DForOutWhenUnconnected=off
  TSphF_B : Outport  Port=4  VectorParamsAs1DForOutWhenUnconnected=off
  TConB : Outport  Port=5  VectorParamsAs1DForOutWhenUnconnected=off
  wires:
  FConB/2(FyConB) -> Divide6/2, Tz in B/2(FyConB), Tx in B/1(FyConB)
  Mux1/1 -> TSphF_B/1
  Divide3/1 -> FConB/4(FAxis)  "FAxis"
  FConB/1(FxConB) -> Ty in B/1(FxConB), Tz in B/1(FxConB), Divide5/2
  FConB/3(FzConB) -> Divide9/2, Ty in B/2(FzConB), Tx in B/2(FzConB)
  Divide4/1 -> FConB/3(FRing), Tz in B/7(FRing)  "FRing"
  Mux/1 -> Divide7/2
  Ff/1 -> Divide4/1, Divide3/1  "Ff abs"
  alpha/1 -> cos1/1, sin1/1
  cos1/1 -> Divide3/2
  sin/1 -> FConB/2(cosazm), Ty in B/3(cosazm), Tz in B/4(cosazm)
  azm/1 -> cos/1, sin/1
  cos/1 -> FConB/1(sinazm), Tz in B/3(sinazm), Tx in B/3(sinazm)
  sin1/1 -> Divide4/2
  rConAxtoCP/1 -> Tx in B/5(rConAxtoCP), Ty in B/5(rConAxtoCP), Tz in B/5(rConAxtoCP)
  rSphtoCP/1 -> Ty in B/6(rSphtoCP), Tz in B/6(rSphtoCP), Tx in B/6(rSphtoCP)
  z/1 -> Ty in B/4(z), Tx in B/4(z)
  Tx in B/1(TxConB) -> Mux/1
  Ty in B/1(TyConB) -> Mux/2
  Tx in B/2(TxSph_B) -> Mux1/1  "Tx_B"
  Ty in B/2(TySph_B) -> Mux1/2  "Ty_B"
  InOut/1 -> [inOut]
  Divide9/1 -> FzConB/1
  Divide5/1 -> FxConB/1
  Divide6/1 -> FyConB/1
  [inOut] -> Divide5/1
  [inOut] -> Divide6/1
  [inOut] -> Divide9/1
  Tz in B/1(TzConB) -> Mux/3
  Tz in B/2(TzSph_B) -> Mux1/3  "Tz_B"
  [inOut] -> Divide7/1
  Divide7/1 -> TConB/1

== system Contact_Forces_Lib/3D/Sphere to Cone Force/Forces/Ff/Resolve Ff/Ff in SphF ==
  FxConB : Inport
  FyConB : Inport  Port=2
  FzConB : Inport  Port=3
  TSphF_B : Inport  Port=4
  R : Inport  Port=5
  Demux : Demux  Outputs=3
  Divide1 : Product  Inputs=/*  Multiplication=Matrix(*)
  Divide3 : Product  Inputs=/*  Multiplication=Matrix(*)
  Gain1 : Gain  Gain=-1
  Mux1 : Mux  Inputs=3
  FySphF : Outport  VectorParamsAs1DForOutWhenUnconnected=off
  FxSphF : Outport  Port=2  VectorParamsAs1DForOutWhenUnconnected=off
  FzSphF : Outport  Port=3  VectorParamsAs1DForOutWhenUnconnected=off
  TSphF : Outport  Port=4  VectorParamsAs1DForOutWhenUnconnected=off
  wires:
  TSphF_B/1 -> Divide1/2
  Demux/3 -> FzSphF/1
  Demux/2 -> FySphF/1
  Demux/1 -> FxSphF/1
  FzConB/1 -> Mux1/3
  FxConB/1 -> Mux1/1
  FyConB/1 -> Mux1/2
  Gain1/1 -> Demux/1
  Mux1/1 -> Divide3/2
  Divide3/1 -> Gain1/1
  R/1 -> Divide3/1, Divide1/1
  Divide1/1 -> TSphF/1

== system Contact_Forces_Lib/3D/Sphere to Tube Force/Forces/Ff/Relative vel at CP/Calculate vRelAxis ==
  rSphtoCP sign : Inport
  wxf : Inport  Port=2
  vzf : Inport  Port=3
  azm : Inport  Port=4
  wyf : Inport  Port=5
  " " : Gain  Gain=-1
  Product4 : Product
  Product5 : Product
  Product6 : Product
  Sum4 : Sum  Inputs=+-
  Sum5 : Sum
  Trigonometric Function1 : Trigonometry
  Trigonometric Function2 : Trigonometry  Operator=cos
  vRelAxis : Outport  VectorParamsAs1DForOutWhenUnconnected=off
  wires:
  " "/1 -> Sum5/2  "wCPy"
  Product6/1 -> " "/1
  wxf/1 -> Product5/1
  Product5/1 -> Sum5/1  "wCPx"
  Trigonometric Function2/1 -> Product6/1
  Sum4/1 -> vRelAxis/1  "vRelAxis"
  vzf/1 -> Sum4/1  "vAxisTra"
  Sum5/1 -> Product4/2  "wCP"
  azm/1 -> Trigonometric Function2/1, Trigonometric Function1/1
  wyf/1 -> Product6/2
  Product4/1 -> Sum4/2  "vAxisRot"
  Trigonometric Function1/1 -> Product5/2
  rSphtoCP sign/1 -> Product4/1

== system Contact_Forces_Lib/3D/Sphere to Tube Force/Forces/Ff/Relative vel at CP/Calculate vRelRing ==
  rad : Inport
  vazm : Inport  Port=2
  wzf : Inport  Port=3
  rSphtoCP sign : Inport  Port=4
  Product1 : Product
  Product2 : Product
  Sum : Sum  Inputs=+-
  Sum1 : Sum  Inputs=+-
  Sum2 : Sum  Inputs=+-
  rCyltoCP : Outport  VectorParamsAs1DForOutWhenUnconnected=off
  vRelRing : Outport  Port=2  VectorParamsAs1DForOutWhenUnconnected=off
  wires:
  Product1/1 -> Sum2/2  "vRingRot"
  Sum2/1 -> vRelRing/1  "vrelRing"
  Sum/1 -> rCyltoCP/1, Product2/2  "rCyltoCP"
  Product2/1 -> Sum2/1  "vRingTra"
  vazm/1 -> Product2/1, Sum1/2
  wzf/1 -> Sum1/1
  rad/1 -> Sum/1
  rSphtoCP sign/1 -> Product1/2, Sum/2
  Sum1/1 -> Product1/1
